simulink model "Controller"  (R2018b)
settings: configuration reference "control_config" (kept outside this file)
values from neighbouring files (symbols this model uses):
  CONTROL_EXPORT = Simulink.Parameter(CONTROL_EXPORT_VALUE)    [controller_model_init.m]
  CONTROL_PARAM = Simulink.Parameter(CONTROL_PARAM_VALUE)    [controller_model_init.m]
undefined symbols (not defined in the file or in its folder): actuator_cmd, CONTROL_CONST, ControlMode, DiscIntNeverNeededParam, PilotMode, timestamp, VehicleStatus, VTOLState
libraries: simulink x31, FMT_Model_Lib x20
(part 3 of 3)

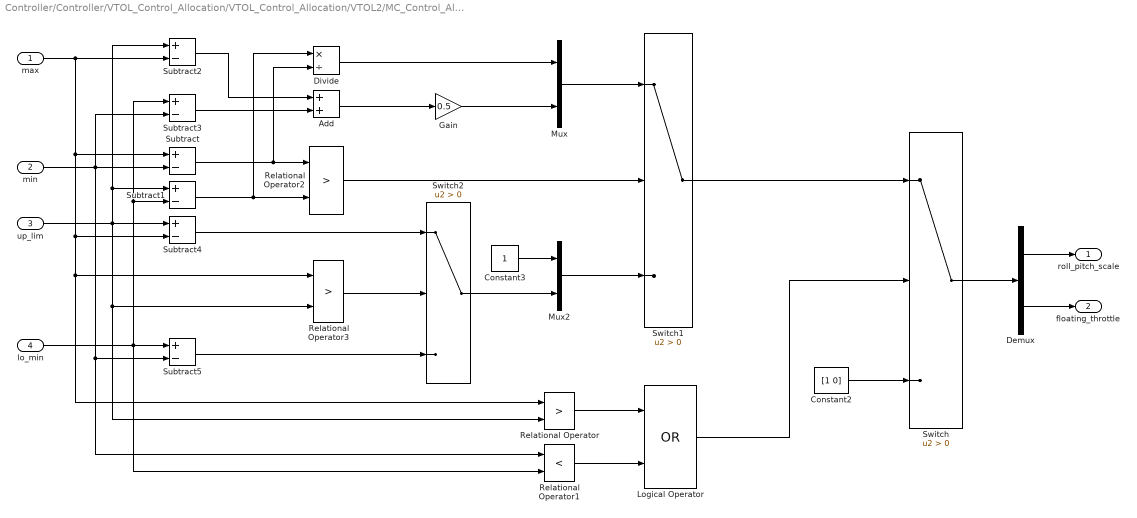
== system Controller/Controller/VTOL_Control_Allocation/VTOL_Control_Allocation/VTOL2/MC_Control_Allocation/P_Q_Remix1 ==
  max : Inport
  min : Inport  Port=2
  up_lim : Inport  Port=3
  lo_min : Inport  Port=4
  Add : Sum
  Constant2 : Constant  Value=[1 0]  OutDataTypeStr=single
  Constant3 : Constant  OutDataTypeStr=single
  Demux : Demux  Outputs=2
  Divide : Product  Inputs=*/
  Gain : Gain  Gain=0.5
  Logical Operator : Logic  Operator=OR  AllPortsSameDT=off  OutDataTypeStr=boolean
  Mux : Mux  Inputs=2
  Mux2 : Mux  Inputs=2
  Relational Operator : RelationalOperator  Operator=>  OutDataTypeStr=boolean  RndMeth=Simplest
  Relational Operator1 : RelationalOperator  Operator=<  OutDataTypeStr=boolean  RndMeth=Simplest
  Relational Operator2 : RelationalOperator  Operator=>  OutDataTypeStr=boolean  RndMeth=Simplest
  Relational Operator3 : RelationalOperator  Operator=>  OutDataTypeStr=boolean  RndMeth=Simplest
  Subtract{,1..5} (6 alike) : Sum  Inputs=+-
  Switch : Switch  Criteria=u2 > Threshold
  Switch1 : Switch  Criteria=u2 > Threshold
  Switch2 : Switch  Criteria=u2 > Threshold
  roll_pitch_scale : Outport
  floating_throttle : Outport  Port=2
  wires:
  max/1 -> Subtract2/2, Subtract/1, Relational Operator3/1, Relational Operator/1, Subtract4/2
  up_lim/1 -> Relational Operator/2, Relational Operator3/2, Subtract2/1, Subtract1/1, Subtract4/1
  min/1 -> Subtract3/2, Subtract/2, Relational Operator1/1, Subtract5/2
  lo_min/1 -> Relational Operator1/2, Subtract3/1, Subtract1/2, Subtract5/1
  Relational Operator/1 -> Logical Operator/1
  Relational Operator1/1 -> Logical Operator/2
  Logical Operator/1 -> Switch/2
  Constant2/1 -> Switch/3
  Subtract/1 -> Relational Operator2/1, Divide/2
  Subtract1/1 -> Relational Operator2/2, Divide/1
  Relational Operator2/1 -> Switch1/2
  Divide/1 -> Mux/1
  Subtract2/1 -> Add/1
  Subtract3/1 -> Add/2
  Add/1 -> Gain/1
  Gain/1 -> Mux/2
  Mux/1 -> Switch1/1
  Relational Operator3/1 -> Switch2/2
  Subtract4/1 -> Switch2/1
  Switch1/1 -> Switch/1
  Switch/1 -> Demux/1
  Demux/1 -> roll_pitch_scale/1
  Demux/2 -> floating_throttle/1
  Switch2/1 -> Mux2/2
  Mux2/1 -> Switch1/3
  Constant3/1 -> Mux2/1
  Subtract5/1 -> Switch2/3

== system Controller/Controller/VTOL_Control_Allocation/VTOL_Control_Allocation/VTOL2/actuator_cmd_routing/Disarm ==
  Bias : Bias  Bias=CONTROL_PARAM.SERVO1_BIAS
  Bias1 : Bias  Bias=CONTROL_PARAM.SERVO2_BIAS
  Bias2 : Bias  Bias=CONTROL_PARAM.SERVO3_BIAS
  Bias3 : Bias  Bias=CONTROL_PARAM.SERVO4_BIAS
  Constant : Constant  Value=1500  OutDataTypeStr=single
  Data Type Conversion : DataTypeConversion  OutDataTypeStr=uint16
  Disarm : Constant  Value=[1000 1000 1000 1000 1000]'  VectorParams1D=off  OutDataTypeStr=single
  Mux : Mux  Inputs=5
  Reshape : Reshape  OutputDimensionality=Column vector (2-D)
  Saturation : Saturate  UpperLimit=2000  LowerLimit=1000
  actuator_cmd : Outport
  wires:
  Disarm/1 -> Mux/1
  Constant/1 -> Bias3/1, Bias2/1, Bias1/1, Bias/1
  Mux/1 -> Reshape/1
  Data Type Conversion/1 -> actuator_cmd/1
  Saturation/1 -> Data Type Conversion/1
  Reshape/1 -> Saturation/1
  Bias/1 -> Mux/2
  Bias1/1 -> Mux/3
  Bias2/1 -> Mux/4
  Bias3/1 -> Mux/5

== system Controller/Controller/VTOL_Control_Allocation/VTOL_Control_Allocation/VTOL2/actuator_cmd_routing/Standby ==
  Bias : Bias  Bias=CONTROL_PARAM.SERVO1_BIAS
  Bias1 : Bias  Bias=CONTROL_PARAM.SERVO2_BIAS
  Bias2 : Bias  Bias=CONTROL_PARAM.SERVO3_BIAS
  Bias3 : Bias  Bias=CONTROL_PARAM.SERVO4_BIAS
  Constant : Constant  Value=1500  OutDataTypeStr=single
  Data Type Conversion : DataTypeConversion  OutDataTypeStr=uint16
  Disarm : Constant  Value=[1150 1150 1150 1150 1000]'  VectorParams1D=off  OutDataTypeStr=single
  Mux : Mux  Inputs=5
  Reshape : Reshape  OutputDimensionality=Column vector (2-D)
  Saturation : Saturate  UpperLimit=2000  LowerLimit=1000
  actuator_cmd : Outport
  wires:
  Bias3/1 -> Mux/5
  Bias2/1 -> Mux/4
  Bias1/1 -> Mux/3
  Bias/1 -> Mux/2
  Reshape/1 -> Saturation/1
  Saturation/1 -> Data Type Conversion/1
  Mux/1 -> Reshape/1
  Constant/1 -> Bias/1, Bias1/1, Bias2/1, Bias3/1
  Disarm/1 -> Mux/1
  Data Type Conversion/1 -> actuator_cmd/1

== system Controller/Controller/FW_Controller/FW_Controller/Attitude_Control/Innerloop_Rate_Control/PI_Control/I_Control ==
  err : Inport
  reset : Inport  Port=2
  Constant : Constant  Value=[0;0;0]  OutDataTypeStr=single
  Discrete-Time Integrator : DiscreteIntegrator  ExternalReset=level  InitialConditionSource=external  SampleTime=-1  LimitOutput=on  UpperSaturationLimit=max_i  LowerSaturationLimit=min_i  ICPrevOutput=DiscIntNeverNeededParam  ICPrevScaledInput=DiscIntNeverNeededParam
  Multiply : Product  OutDataTypeStr=Inherit: Same as first input
  Mux : Mux  Inputs=3
  gain1 : Constant  Value=p_ki  OutDataTypeStr=single
  gain2 : Constant  Value=q_ki  OutDataTypeStr=single
  gain3 : Constant  Value=r_ki  OutDataTypeStr=single
  i_out : Outport
  wires:
  err/1 -> Multiply/2
  gain2/1 -> Mux/2
  gain1/1 -> Mux/1
  gain3/1 -> Mux/3
  reset/1 -> Discrete-Time Integrator/2
  Constant/1 -> Discrete-Time Integrator/3
  Discrete-Time Integrator/1 -> i_out/1
  Mux/1 -> Multiply/1
  Multiply/1 -> Discrete-Time Integrator/1

== system Controller/Controller/FW_Controller/FW_Controller/Attitude_Control/Innerloop_Rate_Control/PI_Control/P_Control ==
  err : Inport
  Multiply : Product  OutDataTypeStr=Inherit: Same as first input
  Mux : Mux  Inputs=3
  gain1 : Constant  Value=p_kp  OutDataTypeStr=single
  gain2 : Constant  Value=q_kp  OutDataTypeStr=single
  gain3 : Constant  Value=r_kp  OutDataTypeStr=single
  p_out : Outport
  wires:
  err/1 -> Multiply/2
  gain2/1 -> Mux/2
  Mux/1 -> Multiply/1
  gain1/1 -> Mux/1
  Multiply/1 -> p_out/1
  gain3/1 -> Mux/3

== system Controller/Controller/FW_Controller/FW_Controller/Attitude_Control/Outloop_Angle_Control/Attitude_Controller/Error ==
  att_cmd : Inport
  INS_Out : Inport  Port=2
  Bus_Select : Subsystem
  Demux : Demux  Outputs=2
  Mux : Mux  Inputs=2
  Pitch Offset : Bias  Bias=CONTROL_PARAM.FW_PITCH_OFFSET
  Saturation : Saturate  UpperLimit=CONTROL_PARAM.FW_ROLL_PITCH_CMD_LIM  LowerLimit=-CONTROL_PARAM.FW_ROLL_PITCH_CMD_LIM
  Sum : Sum  Inputs=|+-
  euler_err_rad : Outport
  wires:
  att_cmd/1 -> Demux/1
  Sum/1 -> euler_err_rad/1  "fw_att_error_B_rad"
  INS_Out/1 -> Bus_Select/1(INS_Out)
  Bus_Select/1(att_est_B_rad) -> Sum/2  "fw_att_est_B_rad"
  Demux/2 -> Pitch Offset/1
  Demux/1 -> Mux/1
  Pitch Offset/1 -> Mux/2
  Mux/1 -> Saturation/1
  Saturation/1 -> Sum/1  "fw_att_cmd_B_rad"

== system Controller/Controller/FW_Controller/FW_Controller/Attitude_Control/Outloop_Angle_Control/Attitude_Controller/P_Controller ==
  error : Inport
  Constant1 : Constant  Value=CONTROL_PARAM.FW_ROLL_P
  Constant2 : Constant  Value=CONTROL_PARAM.FW_PITCH_P
  Multiply : Product
  Mux : Mux  Inputs=2
  u : Outport
  wires:
  Multiply/1 -> u/1
  error/1 -> Multiply/1
  Mux/1 -> Multiply/2
  Constant1/1 -> Mux/1
  Constant2/1 -> Mux/2

== system Controller/Controller/FW_Controller/FW_Controller/Attitude_Control/Outloop_Angle_Control/Heading_Controller/Turning_Coordination ==
  note: avoid small VT generate big pdi_rate_sp
  phi_sp : Inport
  theta_sp : Inport  Port=2
  VT : Inport  Port=3
  Constant : Constant  Value=9.81  OutDataTypeStr=single
  Cos : Trigonometry  Operator=cos
  Divide : Product  Inputs=*/
  Multiply : Product
  Multiply1 : Product
  Saturation : Saturate  UpperLimit=1  LowerLimit=0.2
  Tan : Trigonometry  Operator=tan
  psi_rate_sp : Outport
  wires:
  phi_sp/1 -> Tan/1
  theta_sp/1 -> Cos/1
  Constant/1 -> Divide/1
  VT/1 -> Divide/2
  Tan/1 -> Multiply/1
  Cos/1 -> Multiply/2
  Multiply/1 -> Multiply1/1
  Multiply1/1 -> psi_rate_sp/1
  Divide/1 -> Saturation/1
  Saturation/1 -> Multiply1/2

== system Controller/Controller/MC_Controller/Horizontal_Control/Attitude_Controller/Inner_Loop/ATT_Cmd_Mixer/Backward_Mixer ==
  mc_cmd : Inport
  aux_cmd : Inport  Port=2
  VT : Inport  Port=3
  Constant : Constant  Value=max  OutDataTypeStr=single
  Constant1 : Constant  Value=min  OutDataTypeStr=single
  Constant2 : Constant  OutDataTypeStr=single
  Constant3 : Constant  OutDataTypeStr=single
  Divide : Product  Inputs=*/
  Multiply : Product
  Multiply1 : Product
  Multiply2 : Product
  Saturation3 : Saturate  UpperLimit=max  LowerLimit=min
  Subtract : Sum  Inputs=+-
  Subtract1 : Sum  Inputs=-+
  Sum : Sum  Inputs=-+|
  Sum1 : Sum  Inputs=|++
  mix_rate_cmd : Outport
  wires:
  VT/1 -> Saturation3/1
  Constant/1 -> Subtract/1
  Constant1/1 -> Subtract1/1, Subtract/2
  Subtract/1 -> Divide/2
  Constant2/1 -> Divide/1
  Divide/1 -> Multiply/1
  Saturation3/1 -> Subtract1/2
  Subtract1/1 -> Multiply/2
  Multiply/1 -> Multiply2/1, Sum/1  "aux_gain"
  Constant3/1 -> Sum/2
  Sum/1 -> Multiply1/1  "mc_gain"
  mc_cmd/1 -> Multiply1/2
  aux_cmd/1 -> Multiply2/2
  Multiply2/1 -> Sum1/1
  Multiply1/1 -> Sum1/2
  Sum1/1 -> mix_rate_cmd/1

== system Controller/Controller/MC_Controller/Horizontal_Control/Attitude_Controller/Inner_Loop/ATT_Cmd_Mixer/Fly_Speed ==
  INS_Out : Inport
  Bus Selector2 : BusSelector  OutputSignals=vn,ve,vd
  Bus Selector3 : BusSelector  OutputSignals=quat
  Multiply : Product  Multiplication=Matrix(*)
  Mux : Mux  Inputs=3
  Quaternion To DCM : FMT_Model_Lib/Quaternion/Quaternion To DCM
      settings: SourceProductName=FMT Toolbox
  Selector : Selector  InputPortWidth=3  IndexOptions=Index vector (dialog)  Indices=1  OutputSizes=1
  speed : Outport
  wires:
  Bus Selector3/1 -> Quaternion To DCM/1  "<quat>"
  Multiply/1 -> Selector/1
  Bus Selector2/3 -> Mux/3  "<vd>"
  INS_Out/1 -> Bus Selector3/1, Bus Selector2/1
  Mux/1 -> Multiply/2
  Quaternion To DCM/1 -> Multiply/1
  Bus Selector2/2 -> Mux/2  "<ve>"
  Bus Selector2/1 -> Mux/1  "<vn>"
  Selector/1 -> speed/1  "Vu"

== system Controller/Controller/MC_Controller/Horizontal_Control/Attitude_Controller/Inner_Loop/ATT_Cmd_Mixer/Forward_Mixer ==
  mc_cmd : Inport
  aux_cmd : Inport  Port=2
  VT : Inport  Port=3
  Constant : Constant  Value=max  OutDataTypeStr=single
  Constant1 : Constant  Value=min  OutDataTypeStr=single
  Constant2 : Constant  OutDataTypeStr=single
  Constant3 : Constant  OutDataTypeStr=single
  Constant4 : Constant  OutDataTypeStr=single
  Divide : Product  Inputs=*/
  Gain : Gain  Gain=0  OutDataTypeStr=Inherit: Same as input
  Multiply : Product
  Multiply1 : Product
  Multiply2 : Product
  Mux : Mux  Inputs=3
  Mux1 : Mux  Inputs=3
  Saturation3 : Saturate  UpperLimit=max  LowerLimit=min
  Subtract : Sum  Inputs=+-
  Subtract1 : Sum  Inputs=-+
  Sum : Sum  Inputs=-+|
  Sum1 : Sum  Inputs=|++
  mix_rate_cmd : Outport
  wires:
  Sum1/1 -> mix_rate_cmd/1
  Multiply1/1 -> Sum1/2
  Multiply2/1 -> Sum1/1
  aux_cmd/1 -> Multiply2/2
  mc_cmd/1 -> Multiply1/2
  Sum/1 -> Mux1/3, Gain/1, Mux1/1  "mc_gain"
  Constant3/1 -> Sum/2
  Multiply/1 -> Mux/1, Mux/3, Sum/1  "aux_gain"
  Subtract1/1 -> Multiply/2
  Saturation3/1 -> Subtract1/2
  Divide/1 -> Multiply/1
  Constant2/1 -> Divide/1
  Subtract/1 -> Divide/2
  Constant1/1 -> Subtract/2, Subtract1/1
  Constant/1 -> Subtract/1
  VT/1 -> Saturation3/1
  Constant4/1 -> Mux/2
  Mux/1 -> Multiply2/1
  Gain/1 -> Mux1/2
  Mux1/1 -> Multiply1/1

== system Controller/Controller/MC_Controller/Horizontal_Control/Attitude_Controller/Inner_Loop/Rate_Controller/Error ==
  rate_cmd_radPs : Inport
  INS_Out : Inport  Port=2
  Bus_Select : Subsystem
  First Order LPF : FMT_Model_Lib/Filter/First Order LPF  fc=30
      settings: SourceProductName=FMT Toolbox
  Saturation : Saturate  UpperLimit=pi  LowerLimit=-pi
  Sum : Sum  Inputs=|+-
  rate_err_radPs : Outport
  wires:
  Sum/1 -> Saturation/1  "rate_error_B_radPs"
  rate_cmd_radPs/1 -> Sum/1  "rate_cmd_B_radPs"
  INS_Out/1 -> Bus_Select/1(INS_Out)
  Bus_Select/1(rate_est_radPs) -> Sum/2  "rate_est_B_radPs"
  First Order LPF/1 -> rate_err_radPs/1
  Saturation/1 -> First Order LPF/1

== system Controller/Controller/MC_Controller/Horizontal_Control/Attitude_Controller/Inner_Loop/Rate_Controller/Feedforward_Controller ==
  rate_cmd_radPs : Inport
  DeadZone : Subsystem  mask{th=0.1}
      mask prompts: th "Threshold"
      mask Display: disp('Dead Zone')
  Demux : Demux  Outputs=2
  Gain : Gain  Gain=CONTROL_PARAM.MC_ROLL_RATE_FF
  Gain1 : Gain  Gain=CONTROL_PARAM.MC_PITCH_RATE_FF
  Mux : Mux  Inputs=2
  rate_dot_cmd_B : Outport
  wires:
  rate_cmd_radPs/1 -> DeadZone/1(u)
  Demux/2 -> Gain1/1
  Demux/1 -> Gain/1
  Gain1/1 -> Mux/2
  DeadZone/1(y) -> Demux/1
  Mux/1 -> rate_dot_cmd_B/1
  Gain/1 -> Mux/1

== system Controller/Controller/MC_Controller/Horizontal_Control/Attitude_Controller/Inner_Loop/Rate_Controller/PID_Controller ==
  rate_err_radPs : Inport
  reset : Inport  Port=2
  Add : Sum  Inputs=+++
  D_Control : Subsystem  mask{p_kd=CONTROL_PARAM.MC_ROLL_RATE_D, q_kd=CONTROL_PARAM.MC_PITCH_RATE_D, r_kd=CONTROL_PARAM.MC_YAW_RATE_D, max_d=CONTROL_PARAM.MC_RATE_D_MAX, min_d=CONTROL_PARAM.MC_RATE_D_MIN}
  I_Control : Subsystem  mask{p_ki=CONTROL_PARAM.MC_ROLL_RATE_I, q_ki=CONTROL_PARAM.MC_PITCH_RATE_I, r_ki=CONTROL_PARAM.MC_YAW_RATE_I, max_i=CONTROL_PARAM.MC_RATE_I_MAX, min_i=CONTROL_PARAM.MC_RATE_I_MIN}
  P_Control : Subsystem  mask{p_kp=CONTROL_PARAM.MC_ROLL_RATE_P, q_kp=CONTROL_PARAM.MC_PITCH_RATE_P, r_kp=CONTROL_PARAM.MC_YAW_RATE_P}
  rate_dot_cmd_B : Outport
  wires:
  rate_err_radPs/1 -> P_Control/1(err), I_Control/1(err), D_Control/1(err)
  P_Control/1(p_out) -> Add/1  "torque_p_out"
  I_Control/1(i_out) -> Add/2  "torque_i_out"
  D_Control/1(d_out) -> Add/3  "torque_d_out"
  reset/1 -> I_Control/2(reset), D_Control/2(reset)
  Add/1 -> rate_dot_cmd_B/1

== system Controller/Controller/MC_Controller/Horizontal_Control/Attitude_Controller/Outter_Loop/Attitude_Controller/Error ==
  att_cmd : Inport
  INS_Out : Inport  Port=2
  Bus_Select : Subsystem
  Sum : Sum  Inputs=|+-
  euler_err_rad : Outport
  wires:
  att_cmd/1 -> Sum/1  "att_cmd_B_rad"
  Sum/1 -> euler_err_rad/1  "att_error_B_rad"
  INS_Out/1 -> Bus_Select/1(INS_Out)
  Bus_Select/1(att_est_B_rad) -> Sum/2  "att_est_B_rad"

== system Controller/Controller/MC_Controller/Horizontal_Control/Attitude_Controller/Outter_Loop/Attitude_Controller/Sqrt_Root_Controller ==
  euler_err_rad : Inport
  Constant1 : Constant  Value=CONTROL_PARAM.MC_ROLL_P
  Constant2 : Constant  Value=CONTROL_PARAM.MC_PITCH_P
  Mux : Mux  Inputs=2
  Sqrt_Root_Control : Subsystem  mask{dt=CONTROL_CONST.dt, second_ord_lim=9.5993}
      mask prompts: second_ord_lim "2nd-order lim"
  euler_rate_cmd_radPs : Outport
  wires:
  Sqrt_Root_Control/1(out) -> euler_rate_cmd_radPs/1
  euler_err_rad/1 -> Sqrt_Root_Control/1(error)
  Mux/1 -> Sqrt_Root_Control/2(p)
  Constant1/1 -> Mux/1
  Constant2/1 -> Mux/2

== system Controller/Controller/MC_Controller/Horizontal_Control/Attitude_Controller/Outter_Loop/Signal_Select/Offboard_Signal_Select ==
  FMS_Out : Inport
  att_cmd_in : Inport  Port=2
  Bus Selector1 : BusSelector  OutputSignals=cmd_mask
  Bus Selector2 : BusSelector  OutputSignals=phi_cmd,theta_cmd
  Mux1 : Mux  Inputs=2
  Mux2 : Mux  Inputs=2
  Switch : Switch  Criteria=u2 > Threshold
  cmd_phi valid : simulink/Logic and Bit Operations/Bitwise Operator  logicop=AND  UseBitMask=on  BitMask=bin2dec('1000')  BitMaskRealWorld=Stored Integer
  cmd_theta valid : simulink/Logic and Bit Operations/Bitwise Operator  logicop=AND  UseBitMask=on  BitMask=bin2dec('10000')  BitMaskRealWorld=Stored Integer
  att_cmd_rad : Outport
  wires:
  Switch/1 -> att_cmd_rad/1
  FMS_Out/1 -> Bus Selector2/1, Bus Selector1/1
  Bus Selector1/1 -> cmd_theta valid/1, cmd_phi valid/1  "<cmd_mask>"
  cmd_phi valid/1 -> Mux1/1
  cmd_theta valid/1 -> Mux1/2
  Mux1/1 -> Switch/2
  Bus Selector2/1 -> Mux2/1  "<phi_cmd>"
  Bus Selector2/2 -> Mux2/2  "<theta_cmd>"
  Mux2/1 -> Switch/1
  att_cmd_in/1 -> Switch/3

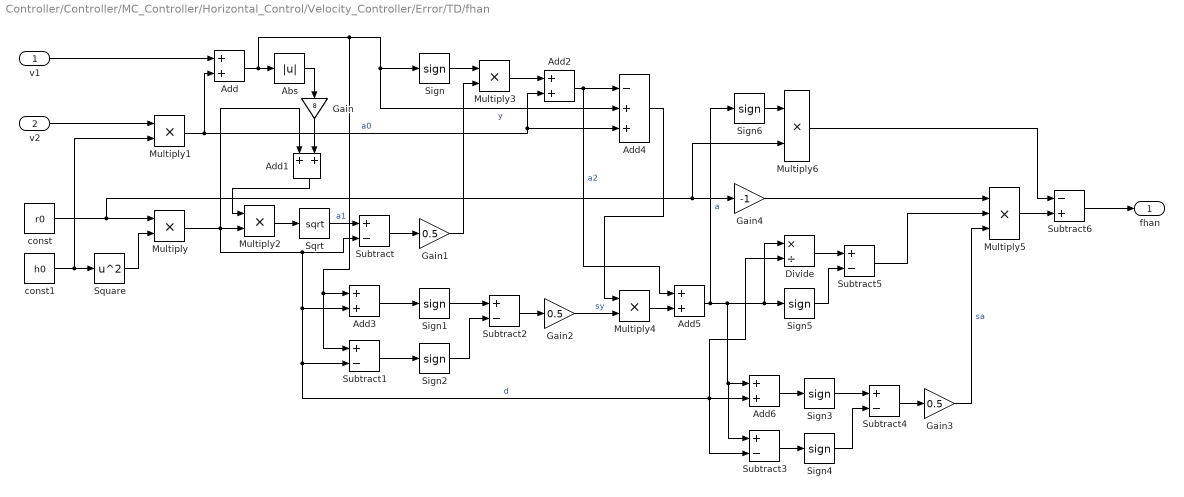
== system Controller/Controller/MC_Controller/Horizontal_Control/Velocity_Controller/Error/TD/fhan  ==
  v1 : Inport
  v2 : Inport  Port=2
  Abs : Abs
  Add{,1..3,5..6} (6 alike) : Sum  OutDataTypeStr=Inherit: Same as first input
  Add4 : Sum  Inputs=-++
  Divide : Product  Inputs=*/
  Gain : Gain  Gain=8
  Gain1 : Gain  Gain=0.5  OutDataTypeStr=Inherit: Same as input
  Gain2 : Gain  Gain=0.5  OutDataTypeStr=Inherit: Same as input
  Gain3 : Gain  Gain=0.5  OutDataTypeStr=Inherit: Same as input
  Gain4 : Gain  Gain=-1  OutDataTypeStr=Inherit: Same as input
  Multiply{,1..3} (4 alike) : Product  OutDataTypeStr=Inherit: Same as first input
  Multiply4 : Product  OutDataTypeStr=single
  Multiply5 : Product  Inputs=3
  Multiply6 : Product  OutDataTypeStr=single
  Sign{,1..6} (7 alike) : Signum
  Sqrt : Sqrt  SaturateOnIntegerOverflow=on
  Square : Math  Operator=square  SaturateOnIntegerOverflow=on
  Subtract{,1..5} (6 alike) : Sum  Inputs=+-  OutDataTypeStr=Inherit: Same as first input
  Subtract6 : Sum  Inputs=-+  OutDataTypeStr=Inherit: Same as first input
  const : Constant  Value=r0  OutDataTypeStr=single
  const1 : Constant  Value=h0  OutDataTypeStr=single
  fhan : Outport
  wires:
  Sign1/1 -> Subtract2/1
  Multiply2/1 -> Sqrt/1
  Square/1 -> Multiply/2
  Gain1/1 -> Multiply3/2
  Multiply6/1 -> Subtract6/1
  Multiply/1 -> Multiply2/2, Add1/1, Add3/2, Subtract1/2, Add6/2, Subtract3/2, Divide/2, Subtract/2  "d"
  Add6/1 -> Sign3/1
  Sign3/1 -> Subtract4/1
  Sign6/1 -> Multiply6/1
  Multiply5/1 -> Subtract6/2
  Gain4/1 -> Multiply5/1
  Subtract4/1 -> Gain3/1
  Add2/1 -> Add5/1, Add4/1  "a2"
  Subtract2/1 -> Gain2/1
  Add/1 -> Abs/1, Sign/1, Add4/2, Add3/1, Subtract1/1  "y"
  Multiply1/1 -> Add/2, Add2/2, Add4/3  "a0"
  Add5/1 -> Add6/1, Subtract3/1, Divide/1, Sign5/1, Sign6/1  "a"
  const1/1 -> Square/1, Multiply1/2
  Multiply4/1 -> Add5/2
  Subtract5/1 -> Multiply5/2
  Add3/1 -> Sign1/1
  const/1 -> Multiply/1, Gain4/1, Multiply6/2
  Gain/1 -> Add1/2
  Multiply3/1 -> Add2/1
  Divide/1 -> Subtract5/1
  Subtract1/1 -> Sign2/1
  Add1/1 -> Multiply2/1
  Subtract3/1 -> Sign4/1
  Sqrt/1 -> Subtract/1  "a1"
  Sign5/1 -> Subtract5/2
  Add4/1 -> Multiply4/1
  Abs/1 -> Gain/1
  Sign4/1 -> Subtract4/2
  Sign2/1 -> Subtract2/2
  Subtract6/1 -> fhan/1
  Subtract/1 -> Gain1/1
  Gain3/1 -> Multiply5/3  "sa"
  v2/1 -> Multiply1/1
  Gain2/1 -> Multiply4/2  "sy"
  Sign/1 -> Multiply3/1
  v1/1 -> Add/1

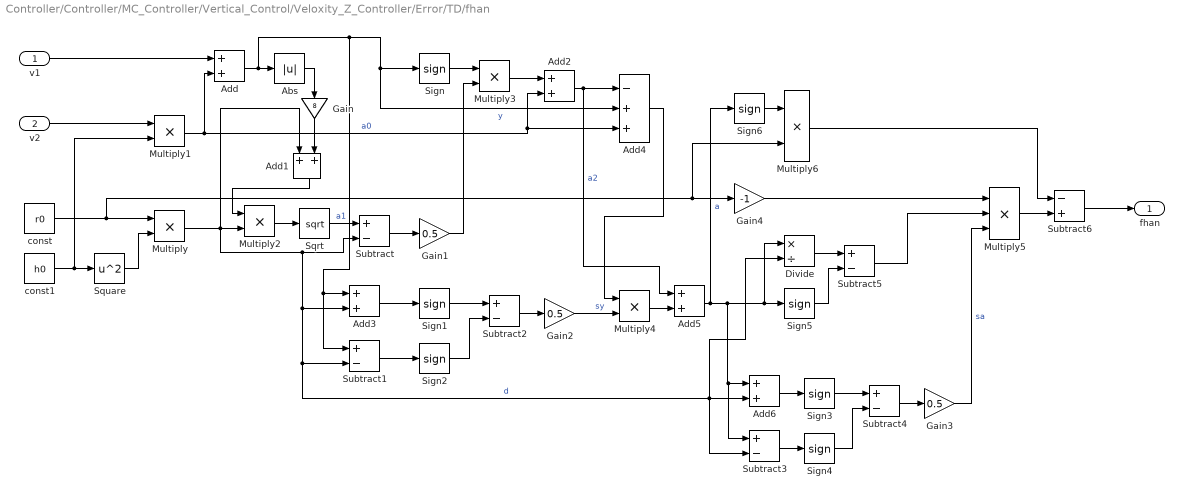
== system Controller/Controller/MC_Controller/Vertical_Control/Veloxity_Z_Controller/Error/TD/fhan  ==
  v1 : Inport
  v2 : Inport  Port=2
  Abs : Abs
  Add{,1..3,5..6} (6 alike) : Sum  OutDataTypeStr=Inherit: Same as first input
  Add4 : Sum  Inputs=-++
  Divide : Product  Inputs=*/
  Gain : Gain  Gain=8
  Gain1 : Gain  Gain=0.5  OutDataTypeStr=Inherit: Same as input
  Gain2 : Gain  Gain=0.5  OutDataTypeStr=Inherit: Same as input
  Gain3 : Gain  Gain=0.5  OutDataTypeStr=Inherit: Same as input
  Gain4 : Gain  Gain=-1  OutDataTypeStr=Inherit: Same as input
  Multiply{,1..3} (4 alike) : Product  OutDataTypeStr=Inherit: Same as first input
  Multiply4 : Product  OutDataTypeStr=single
  Multiply5 : Product  Inputs=3
  Multiply6 : Product  OutDataTypeStr=single
  Sign{,1..6} (7 alike) : Signum
  Sqrt : Sqrt  SaturateOnIntegerOverflow=on
  Square : Math  Operator=square  SaturateOnIntegerOverflow=on
  Subtract{,1..5} (6 alike) : Sum  Inputs=+-  OutDataTypeStr=Inherit: Same as first input
  Subtract6 : Sum  Inputs=-+  OutDataTypeStr=Inherit: Same as first input
  const : Constant  Value=r0  OutDataTypeStr=single
  const1 : Constant  Value=h0  OutDataTypeStr=single
  fhan : Outport
  wires:
  Sign1/1 -> Subtract2/1
  Multiply2/1 -> Sqrt/1
  Square/1 -> Multiply/2
  Gain1/1 -> Multiply3/2
  Multiply6/1 -> Subtract6/1
  Multiply/1 -> Multiply2/2, Add1/1, Add3/2, Subtract1/2, Add6/2, Subtract3/2, Divide/2, Subtract/2  "d"
  Add6/1 -> Sign3/1
  Sign3/1 -> Subtract4/1
  Sign6/1 -> Multiply6/1
  Multiply5/1 -> Subtract6/2
  Gain4/1 -> Multiply5/1
  Subtract4/1 -> Gain3/1
  Add2/1 -> Add5/1, Add4/1  "a2"
  Subtract2/1 -> Gain2/1
  Add/1 -> Abs/1, Sign/1, Add4/2, Add3/1, Subtract1/1  "y"
  Multiply1/1 -> Add/2, Add2/2, Add4/3  "a0"
  Add5/1 -> Add6/1, Subtract3/1, Divide/1, Sign5/1, Sign6/1  "a"
  const1/1 -> Square/1, Multiply1/2
  Multiply4/1 -> Add5/2
  Subtract5/1 -> Multiply5/2
  Add3/1 -> Sign1/1
  const/1 -> Multiply/1, Gain4/1, Multiply6/2
  Gain/1 -> Add1/2
  Multiply3/1 -> Add2/1
  Divide/1 -> Subtract5/1
  Subtract1/1 -> Sign2/1
  Add1/1 -> Multiply2/1
  Subtract3/1 -> Sign4/1
  Sqrt/1 -> Subtract/1  "a1"
  Sign5/1 -> Subtract5/2
  Add4/1 -> Multiply4/1
  Abs/1 -> Gain/1
  Sign4/1 -> Subtract4/2
  Sign2/1 -> Subtract2/2
  Subtract6/1 -> fhan/1
  Subtract/1 -> Gain1/1
  Gain3/1 -> Multiply5/3  "sa"
  v2/1 -> Multiply1/1
  Gain2/1 -> Multiply4/2  "sy"
  Sign/1 -> Multiply3/1
  v1/1 -> Add/1

== system Controller/Controller/FW_Controller/FW_Controller/Attitude_Control/Outloop_Angle_Control/Attitude_Controller/Error/Bus_Select ==
  INS_Out : Inport
  Bus Selector1 : BusSelector  OutputSignals=phi,theta
  Mux1 : Mux  Inputs=2
  att_est_B_rad : Outport
  wires:
  Bus Selector1/2 -> Mux1/2  "<theta>"
  Bus Selector1/1 -> Mux1/1  "<phi>"
  Mux1/1 -> att_est_B_rad/1
  INS_Out/1 -> Bus Selector1/1

== system Controller/Controller/MC_Controller/Horizontal_Control/Attitude_Controller/Inner_Loop/Rate_Controller/Error/Bus_Select ==
  INS_Out : Inport
  Bus Selector1 : BusSelector  OutputSignals=p,q,r
  Mux1 : Mux  Inputs=3
  rate_est_radPs : Outport
  wires:
  Bus Selector1/1 -> Mux1/1  "<p>"
  Bus Selector1/3 -> Mux1/3  "<r>"
  Bus Selector1/2 -> Mux1/2  "<q>"
  Mux1/1 -> rate_est_radPs/1
  INS_Out/1 -> Bus Selector1/1

== system Controller/Controller/MC_Controller/Horizontal_Control/Attitude_Controller/Inner_Loop/Rate_Controller/Feedforward_Controller/DeadZone ==
  u : Inport
  Dead Zone : DeadZone  LowerValue=-th  UpperValue=th  SaturateOnIntegerOverflow=on
  Gain : Gain  Gain=1/(1-th)
  y : Outport
  wires:
  Gain/1 -> y/1
  Dead Zone/1 -> Gain/1
  u/1 -> Dead Zone/1

== system Controller/Controller/MC_Controller/Horizontal_Control/Attitude_Controller/Inner_Loop/Rate_Controller/PID_Controller/D_Control ==
  err : Inport
  reset : Inport  Port=2
  DT Filter : FMT_Model_Lib/Filter/DT Filter  fc=30
      settings: SourceProductName=FMT Toolbox
  Multiply : Product  OutDataTypeStr=Inherit: Same as first input
  Mux : Mux  Inputs=3
  Saturation : Saturate  UpperLimit=max_d  LowerLimit=min_d
  gain1 : Constant  Value=p_kd  OutDataTypeStr=single
  gain2 : Constant  Value=q_kd  OutDataTypeStr=single
  gain3 : Constant  Value=r_kd  OutDataTypeStr=single
  d_out : Outport
  wires:
  err/1 -> DT Filter/1
  gain2/1 -> Mux/2
  gain1/1 -> Mux/1
  Multiply/1 -> Saturation/1
  gain3/1 -> Mux/3
  Saturation/1 -> d_out/1
  reset/1 -> DT Filter/2
  Mux/1 -> Multiply/1
  DT Filter/1 -> Multiply/2

== system Controller/Controller/MC_Controller/Horizontal_Control/Attitude_Controller/Inner_Loop/Rate_Controller/PID_Controller/I_Control ==
  err : Inport
  reset : Inport  Port=2
  Constant : Constant  Value=[0;0;0]  OutDataTypeStr=single
  Discrete-Time Integrator : DiscreteIntegrator  ExternalReset=level  InitialConditionSource=external  SampleTime=-1  LimitOutput=on  UpperSaturationLimit=max_i  LowerSaturationLimit=min_i  ICPrevOutput=DiscIntNeverNeededParam  ICPrevScaledInput=DiscIntNeverNeededParam
  Multiply : Product  OutDataTypeStr=Inherit: Same as first input
  Mux : Mux  Inputs=3
  gain1 : Constant  Value=p_ki  OutDataTypeStr=single
  gain2 : Constant  Value=q_ki  OutDataTypeStr=single
  gain3 : Constant  Value=r_ki  OutDataTypeStr=single
  i_out : Outport
  wires:
  err/1 -> Multiply/2
  gain2/1 -> Mux/2
  gain1/1 -> Mux/1
  gain3/1 -> Mux/3
  reset/1 -> Discrete-Time Integrator/2
  Constant/1 -> Discrete-Time Integrator/3
  Discrete-Time Integrator/1 -> i_out/1
  Mux/1 -> Multiply/1
  Multiply/1 -> Discrete-Time Integrator/1

== system Controller/Controller/MC_Controller/Horizontal_Control/Attitude_Controller/Inner_Loop/Rate_Controller/PID_Controller/P_Control ==
  err : Inport
  Multiply : Product  OutDataTypeStr=Inherit: Same as first input
  Mux : Mux  Inputs=3
  gain1 : Constant  Value=p_kp  OutDataTypeStr=single
  gain2 : Constant  Value=q_kp  OutDataTypeStr=single
  gain3 : Constant  Value=r_kp  OutDataTypeStr=single
  p_out : Outport
  wires:
  err/1 -> Multiply/2
  gain2/1 -> Mux/2
  Mux/1 -> Multiply/1
  gain1/1 -> Mux/1
  Multiply/1 -> p_out/1
  gain3/1 -> Mux/3

== system Controller/Controller/MC_Controller/Horizontal_Control/Attitude_Controller/Outter_Loop/Attitude_Controller/Error/Bus_Select ==
  INS_Out : Inport
  Bus Selector1 : BusSelector  OutputSignals=phi,theta
  Mux1 : Mux  Inputs=2
  att_est_B_rad : Outport
  wires:
  Bus Selector1/2 -> Mux1/2  "<theta>"
  Bus Selector1/1 -> Mux1/1  "<phi>"
  Mux1/1 -> att_est_B_rad/1
  INS_Out/1 -> Bus Selector1/1

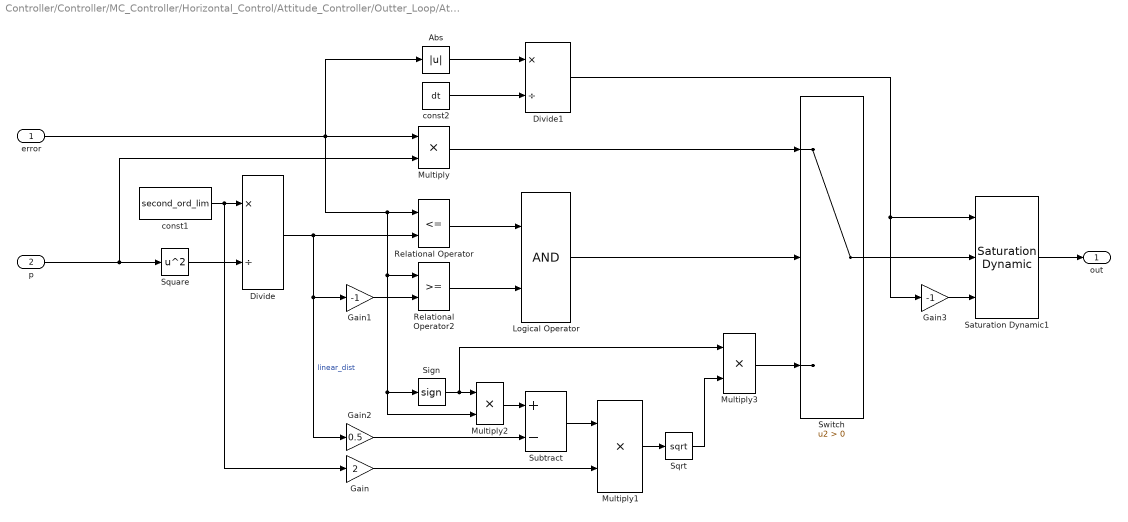
== system Controller/Controller/MC_Controller/Horizontal_Control/Attitude_Controller/Outter_Loop/Attitude_Controller/Sqrt_Root_Controller/Sqrt_Root_Control ==
  error : Inport
  p : Inport  Port=2
  Abs : Abs
  Divide : Product  Inputs=*/
  Divide1 : Product  Inputs=*/
  Gain : Gain  Gain=2  OutDataTypeStr=Inherit: Same as input
  Gain1 : Gain  Gain=-1  OutDataTypeStr=Inherit: Same as input
  Gain2 : Gain  Gain=0.5  OutDataTypeStr=Inherit: Same as input
  Gain3 : Gain  Gain=-1  OutDataTypeStr=Inherit: Same as input
  Logical Operator : Logic  AllPortsSameDT=off  OutDataTypeStr=boolean
  Multiply{,1..3} (4 alike) : Product
  Relational Operator : RelationalOperator  Operator=<=  OutDataTypeStr=boolean  RndMeth=Simplest
  Relational Operator2 : RelationalOperator  OutDataTypeStr=boolean  RndMeth=Simplest
  Saturation Dynamic1 : simulink/Discontinuities/Saturation Dynamic  OutMin=[]  OutMax=[]  OutDataTypeStr=Inherit: Same as second input  OutDataType=fixdt(1, 16)  OutScaling=2^-10  DoSatur=off
  Sign : Signum
  Sqrt : Sqrt  SaturateOnIntegerOverflow=on
  Square : Math  Operator=square  SaturateOnIntegerOverflow=on
  Subtract : Sum  Inputs=+-
  Switch : Switch  Criteria=u2 > Threshold
  const1 : Constant  Value=second_ord_lim  OutDataTypeStr=single
  const2 : Constant  Value=dt  OutDataTypeStr=single
  out : Outport
  wires:
  p/1 -> Multiply/2, Square/1
  const1/1 -> Gain/1, Divide/1
  Square/1 -> Divide/2
  Divide/1 -> Gain2/1, Gain1/1, Relational Operator/2  "linear_dist"
  error/1 -> Abs/1, Multiply/1, Multiply2/2, Sign/1, Relational Operator2/1, Relational Operator/1
  Relational Operator/1 -> Logical Operator/1
  Multiply/1 -> Switch/1
  Switch/1 -> Saturation Dynamic1/2
  Multiply3/1 -> Switch/3
  Gain/1 -> Multiply1/2
  Gain1/1 -> Relational Operator2/2
  Relational Operator2/1 -> Logical Operator/2
  Logical Operator/1 -> Switch/2
  Gain2/1 -> Subtract/2
  Sign/1 -> Multiply3/1, Multiply2/1
  Multiply2/1 -> Subtract/1
  Subtract/1 -> Multiply1/1
  Multiply1/1 -> Sqrt/1
  Sqrt/1 -> Multiply3/2
  Saturation Dynamic1/1 -> out/1
  Abs/1 -> Divide1/1
  const2/1 -> Divide1/2
  Divide1/1 -> Gain3/1, Saturation Dynamic1/1
  Gain3/1 -> Saturation Dynamic1/3

== matlab function Controller/VTOL_Control_Allocation/VTOL_Control_Allocation/VTOL2/MC_Control_Allocation/R_Remix ==
  data: floating_yaw output; motor_out input; up_lim input; lo_lim input
function floating_yaw = fcn(motor_out, up_lim, lo_lim)

min = single(100);
max = single(-100);
min_index = 0;
max_index = 0;

for i = 1 : 4
    if motor_out(i) < min
       min = motor_out(i);
       min_index = i;
    end
    
    if motor_out(i) > max
       max = motor_out(i);
       max_index = i;
    end
end

if max > up_lim || min < lo_lim
    if (max - up_lim) > (lo_lim - min)
        overrun = up_lim - max;
        if max_index == 3 || max_index == 4
            overrun = -overrun;
        end
    else
        overrun =  lo_lim - min;
        if min_index == 3 || min_index == 4
            overrun = -overrun;
        end
    end
    % we assume effective matrix for yaw is [1 1 -1 -1]
    floating_yaw = single([overrun; overrun; -overrun; -overrun]);
else
    floating_yaw = single(zeros(4,1));
end

== matlab function Controller/VTOL_Control_Allocation/VTOL_Control_Allocation/VTOL1/MC_Control_Allocation/R_Remix ==
  data: floating_yaw output; motor_out input; up_lim input; lo_lim input
function floating_yaw = fcn(motor_out, up_lim, lo_lim)

min = single(100);
max = single(-100);
min_index = 0;
max_index = 0;

for i = 1 : 4
    if motor_out(i) < min
       min = motor_out(i);
       min_index = i;
    end
    
    if motor_out(i) > max
       max = motor_out(i);
       max_index = i;
    end
end

if max > up_lim || min < lo_lim
    if (max - up_lim) > (lo_lim - min)
        overrun = up_lim - max;
        if max_index == 3 || max_index == 4
            overrun = -overrun;
        end
    else
        overrun =  lo_lim - min;
        if min_index == 3 || min_index == 4
            overrun = -overrun;
        end
    end
    % we assume effective matrix for yaw is [1 1 -1 -1]
    floating_yaw = single([overrun; overrun; -overrun; -overrun]);
else
    floating_yaw = single(zeros(4,1));
end
